simulink model "Audio_Demo"  (R2026b)
settings: Solver=FixedStepDiscrete  StartTime=0  StopTime=0  FixedStep=1
InitFcn:
  | addpath(fileparts(get_param('Audio_Demo','FileName'))); setup_model('Audio_Demo');
values from neighbouring files (symbols this model uses):
  q = figure('Theme','light','Color','white','Name',[caseId ' quantization error'],      'Tag','JesherDemo','Position',[100 100 1100 450])    [make_plots.m]
undefined symbols (not defined in the file or in its folder): bypassQuantizer, filteredIndices, inputFrame, interpolationWeight, lowerIndices, p, quantMax, quantMin, quantStep, reconstructionTail, referenceAudio, referenceIndices, upperIndices, useFilter
libraries: dspmlti4 x2
settings Model: Creator=jeshe  LastModifiedBy=jeshe
settings DataIOCC: SaveOutput=off  SaveTime=off  SignalLogging=off

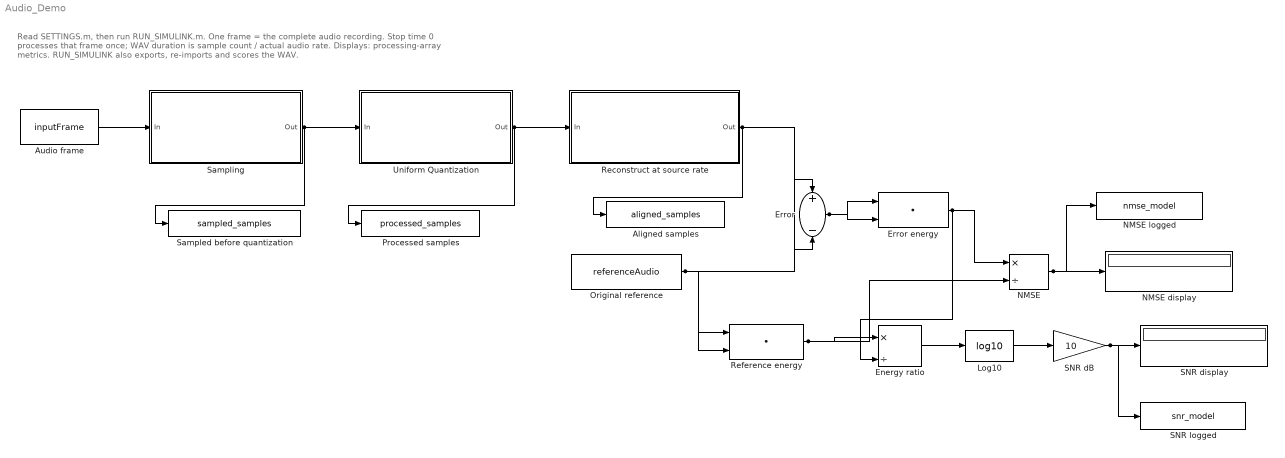
== system Audio_Demo ==
  note: Read SETTINGS.m, then run RUN_SIMULINK.m. One frame = the complete audio recording.
      | Stop time 0 processes that frame once; WAV duration is sample count / actual audio rate.
      | Displays: processing-array metrics. RUN_SIMULINK also exports, re-imports and scores the WAV.
  Aligned samples : ToWorkspace  VariableName=aligned_samples  SampleTime=-1
  Audio frame : Constant  Value=inputFrame  VectorParams1D=off  SampleTime=1
  Energy ratio : Product  Inputs=*/
  Error : Sum  Inputs=+-
  Error energy : DotProduct  OutDataTypeStr=Inherit: Inherit via internal rule
  Log10 : Math  Operator=log10
  NMSE : Product  Inputs=*/
  NMSE display : Display
  NMSE logged : ToWorkspace  VariableName=nmse_model  SampleTime=-1
  Original reference : Constant  Value=referenceAudio  VectorParams1D=off  SampleTime=1
  Processed samples : ToWorkspace  VariableName=processed_samples  SampleTime=-1
  Reconstruct at source rate : Subsystem
  Reference energy : DotProduct  OutDataTypeStr=Inherit: Inherit via internal rule
  SNR dB : Gain  Gain=10
  SNR display : Display
  SNR logged : ToWorkspace  VariableName=snr_model  SampleTime=-1
  Sampled before quantization : ToWorkspace  VariableName=sampled_samples  SampleTime=-1
  Sampling : Subsystem
  Uniform Quantization : Subsystem
  wires:
  Audio frame/1 -> Sampling/1(In)
  Sampling/1(Out) -> Uniform Quantization/1(In), Sampled before quantization/1
  Uniform Quantization/1(Out) -> Reconstruct at source rate/1(In), Processed samples/1
  Reconstruct at source rate/1(Out) -> Aligned samples/1, Error/2
  Original reference/1 -> Error/1, Reference energy/1, Reference energy/2
  Error/1 -> Error energy/1, Error energy/2
  Error energy/1 -> NMSE/1, Energy ratio/2
  Reference energy/1 -> NMSE/2, Energy ratio/1
  Energy ratio/1 -> Log10/1
  Log10/1 -> SNR dB/1
  NMSE/1 -> NMSE display/1, NMSE logged/1
  SNR dB/1 -> SNR display/1, SNR logged/1

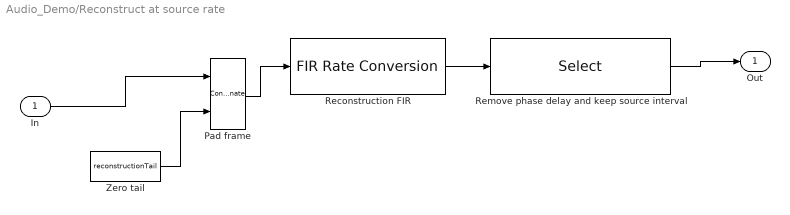
== system Audio_Demo/Reconstruct at source rate ==
  In : Inport
  Pad frame : Concatenate  Mode=Multidimensional array
  Reconstruction FIR : dspmlti4/FIR Rate Conversion  FilterSource=Dialog parameters  L=q  h=reconstructionCoefficients  M=p  FilterObject=FRC  rateMode=Enforce single-rate processing  AllowArbitraryInputLength=off  roundingMode=Floor  overflowMode=off  firstCoeffDataTypeStr=Inherit: Same word length as input  firstCoeffMin=[]  firstCoeffMax=[]  firstCoeffLastDataTypeStr=Inherit: Same word length as input  outputDataTypeStr=Inherit: Same as accumulator  outputMin=[]  outputMax=[]  outputLastDataTypeStr=Inherit: Same as accumulator
  Remove phase delay and keep source interval : Selector  NumberOfDimensions=2  InputPortWidth=3  IndexOptions=Index vector (dialog),Select all  Indices=referenceIndices,1  OutputSizes=1
  Zero tail : Constant  Value=reconstructionTail  VectorParams1D=off  SampleTime=1
  Out : Outport
  wires:
  In/1 -> Pad frame/1
  Zero tail/1 -> Pad frame/2
  Pad frame/1 -> Reconstruction FIR/1
  Reconstruction FIR/1 -> Remove phase delay and keep source interval/1
  Remove phase delay and keep source interval/1 -> Out/1

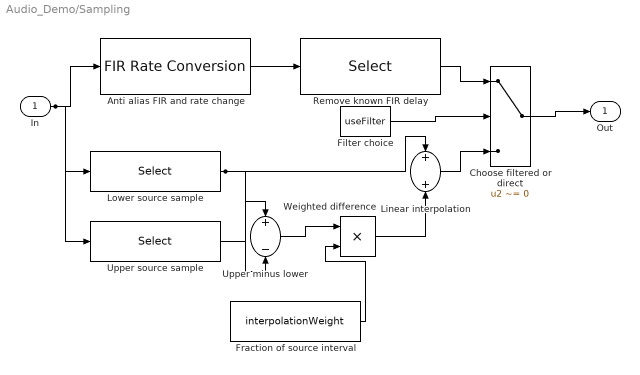
== system Audio_Demo/Sampling ==
  In : Inport
  Anti alias FIR and rate change : dspmlti4/FIR Rate Conversion  FilterSource=Dialog parameters  L=p  h=filterCoefficients  M=q  FilterObject=FRC  rateMode=Enforce single-rate processing  AllowArbitraryInputLength=off  roundingMode=Floor  overflowMode=off  firstCoeffDataTypeStr=Inherit: Same word length as input  firstCoeffMin=[]  firstCoeffMax=[]  firstCoeffLastDataTypeStr=Inherit: Same word length as input  outputDataTypeStr=Inherit: Same as accumulator  outputMin=[]  outputMax=[]  outputLastDataTypeStr=Inherit: Same as accumulator
  Choose filtered or direct : Switch  Criteria=u2 ~= 0  SaturateOnIntegerOverflow=off  InputSameDT=off
  Filter choice : Constant  Value=useFilter  VectorParams1D=off  SampleTime=1
  Fraction of source interval : Constant  Value=interpolationWeight  VectorParams1D=off  SampleTime=1
  Linear interpolation : Sum
  Lower source sample : Selector  NumberOfDimensions=2  InputPortWidth=3  IndexOptions=Index vector (dialog),Select all  Indices=lowerIndices,1  OutputSizes=1
  Remove known FIR delay : Selector  NumberOfDimensions=2  InputPortWidth=3  IndexOptions=Index vector (dialog),Select all  Indices=filteredIndices,1  OutputSizes=1
  Upper minus lower : Sum  Inputs=+-
  Upper source sample : Selector  NumberOfDimensions=2  InputPortWidth=3  IndexOptions=Index vector (dialog),Select all  Indices=upperIndices,1  OutputSizes=1
  Weighted difference : Product
  Out : Outport
  wires:
  In/1 -> Anti alias FIR and rate change/1, Lower source sample/1, Upper source sample/1
  Anti alias FIR and rate change/1 -> Remove known FIR delay/1
  Upper source sample/1 -> Upper minus lower/1
  Lower source sample/1 -> Upper minus lower/2, Linear interpolation/1
  Upper minus lower/1 -> Weighted difference/1
  Fraction of source interval/1 -> Weighted difference/2
  Weighted difference/1 -> Linear interpolation/2
  Remove known FIR delay/1 -> Choose filtered or direct/1
  Filter choice/1 -> Choose filtered or direct/2
  Linear interpolation/1 -> Choose filtered or direct/3
  Choose filtered or direct/1 -> Out/1

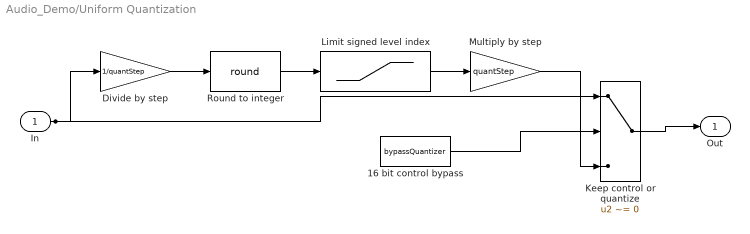
== system Audio_Demo/Uniform Quantization ==
  In : Inport
  16 bit control bypass : Constant  Value=bypassQuantizer  VectorParams1D=off  SampleTime=1
  Divide by step : Gain  Gain=1/quantStep
  Keep control or quantize : Switch  Criteria=u2 ~= 0  SaturateOnIntegerOverflow=off  InputSameDT=off
  Limit signed level index : Saturate  UpperLimit=quantMax  LowerLimit=quantMin
  Multiply by step : Gain  Gain=quantStep
  Round to integer : Rounding  Operator=round
  Out : Outport
  wires:
  In/1 -> Divide by step/1, Keep control or quantize/1
  Divide by step/1 -> Round to integer/1
  Round to integer/1 -> Limit signed level index/1
  Limit signed level index/1 -> Multiply by step/1
  16 bit control bypass/1 -> Keep control or quantize/2
  Multiply by step/1 -> Keep control or quantize/3
  Keep control or quantize/1 -> Out/1
